simulink model "Communication_rate_control"  (R2025a)
settings: Solver=VariableStepAuto  StartTime=0.0  StopTime=30  RelTol=1e-3
InitFcn:
  | %% Simulation parameters and waypoint trajectory
  | % Initial drone positions.
  | init_0=[0;0;0];
  | d_s=4;
  | init_1=init_0+d_s*[-1;0.1;0];
  | init_2=init_0+d_s*[0.3;-2;0];
  | init_3=init_0+d_s*[0.2;3;0];
  | init_4=init_0+d_s*[4;0.4;0];
  | 
  | Threshold = 1000*ones(45,1);
  | for i=1:9:37
  |     Threshold(i:i+2)=10;
  | end
  | gain_2=1;
  | 
  | % PID controller gains.
  | PID_p=20;
  | PID_i=50;
  | PID_d=0;
  | 
  | % Router queues and background traffic.
  | router_buffer=50;
  | router_bandwith=25;
  | router_init_queue=[2,0,0,0,0];
  | traffic_mean=20;
  | traffic_variance=1;
  | 
  | 
  | % Desired formation offsets.
  | init_f_0=[0;0;0];
  | d_f=1;
  | init_f_1=init_0+d_f*[-1;0;0];
  | init_f_2=init_0+d_f*[0;-1;0];
  | init_f_3=init_0+d_f*[0;1;0];
  | init_f_4=init_0+d_f*[1;0;0];
  | 
  | % Quadrotor mass and inertia.
  | mass = 1.2;
  | Ib   = diag([1.2416 1.2416 2*1.2416]);
  | 
  | % Time grid and waypoint trajectory.
  | Ts        = 0.001;
  | ttot      = 20;
  | tdead     = 10;
  | totalTime = ttot + tdead;
  | Nsamples  = 3000;
  | t_sample  = linspace(0, totalTime, Nsamples);
  | t=t_sample;
  | waypoints = [ ...
  |              0  0 -2 0;
  |              3  4 -5 0;
  |              2  1 -8 0;
  |              0 0 -20 0];
  | 
  | M    = size(waypoints,1);
  | t_wp = linspace(0, ttot, M);
  | 
  | p_d      = zeros(4, Nsamples);
  | dot_p_d  = zeros(4, Nsamples);
  | ddot_p_d = zeros(4, Nsamples);
  | 
  | idx_traj = t_sample <= ttot;
  | t_active = t_sample(idx_traj);
  | 
  | % Build position and yaw splines with zero endpoint velocities.
  | for dim = 1:4
  |     pp  = spline(t_wp, [0, waypoints(:,dim)&apos;, 0]);
  |     pp1 = fnder(pp,1);
  |     pp2 = fnder(pp,2);
  | 
  |     p_d(dim,    idx_traj) = ppval(pp,  t_active);
  |     dot_p_d(dim,idx_traj) = ppval(pp1, t_active);
  |     ddot_p_d(dim,idx_traj)= ppval(pp2, t_active);
  | end
  | 
  | % Hold the final waypoint after the maneuver.
  | last_wp_idx = M;
  | p_d(:, ~idx_traj)      = repmat(waypoints(last_wp_idx,:)&apos;, 1, sum(~idx_traj));
  | dot_p_d(:, ~idx_traj)  = 0;
  | ddot_p_d(:, ~idx_traj) = 0;
  | 
  | % Reference signals used by the Simulink blocks.
  | csi_d      = p_d(1:3,:);
  | psi_d      = p_d(4,:);
  | 
  | dot_csi_d  = dot_p_d(1:3,:);
  | ddot_csi_d = ddot_p_d(1:3,:);
  | dot_psi_d  = dot_p_d(4,:);
  | ddot_psi_d = ddot_p_d(4,:);
  | 
  | pos_0     = waypoints(1,1:3);
  | lin_vel_0 = [0 0 0];
  | w_bb_0    = [0 0 0];
undefined symbols (not defined in the file): A_diacenza, DiscIntNeverNeededParam, K, L
libraries: dspsigops x10, robotcorelib x5, slpidlib x5, dspstat3 x5, uavutilslib x1
(part 1 of 3)
settings Model: Creator=fabioruggiero  LastModifiedBy=Giammo
settings ModelReferenceCC: EnableRefExpFcnMdlSchedulingChecks=on
settings RTWCC: GPUComputeCapability=3.5

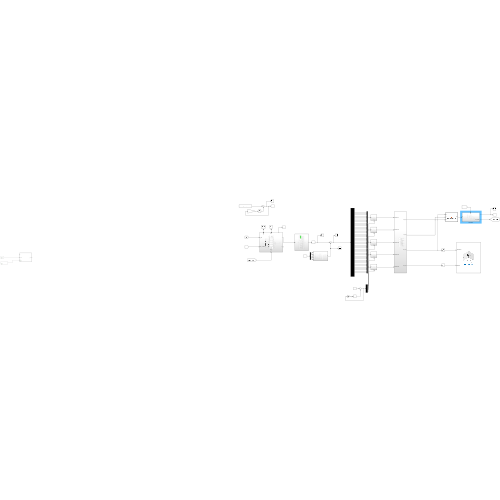
[thumbnail: Simulink's stored preview of the top-level diagram]
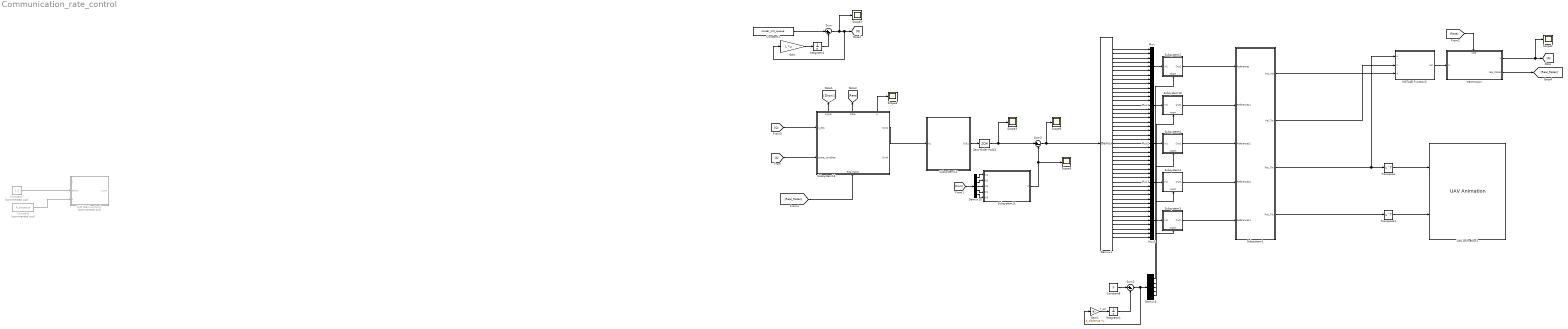
== system Communication_rate_control ==
  Constant : Constant  Commented=on  Value=A_diacenza
  Constant1 : Constant  Value=router_init_queue
  Constant7 : Constant  Commented=on  Value=1.5
  Constant8 : Constant  Value=0
  Demux1 : Demux  Outputs=45
  Demux10 : Demux  Outputs=5
  Demux9 : Demux  Outputs=5
  From : From
  Gain : Gain  Gain=L  Multiplication=Matrix(K*u)
  Gain1 : Gain  Gain=A_diacenza  Multiplication=Matrix(K*u)
  Goto : Goto
  Integrator1 : Integrator
  Integrator2 : Integrator
  MATLAB Function2 : MATLAB Function  TreatAsAtomicUnit=on
  MATLAB Function3 : MATLAB Function  Commented=on  TreatAsAtomicUnit=on
  Mux{,1..3,5} (5 alike) : Mux  Inputs=9
  Scope{1..6} (6 alike) : Scope
      Scope1 settings: ActiveDisplayYMinimum=-19.039927656557538  ActiveDisplayYMaximum=17.096275567841861  DataLoggingVariableName=ScopeData33
      Scope2 settings: ActiveDisplayYMinimum=-0.80480947223759247  ActiveDisplayYMaximum=7.2432852501383342  DataLoggingVariableName=ScopeData34
      Scope3 settings: ActiveDisplayYMinimum=-143.81794768951772  ActiveDisplayYMaximum=72.930943180534939  DataLoggingVariableName=ScopeData22
      Scope4 settings: ActiveDisplayYMinimum=-1  ActiveDisplayYMaximum=1  DataLoggingVariableName=ScopeData10
      Scope5 settings: ActiveDisplayYMinimum=-31.295142586026412  ActiveDisplayYMaximum=31.13864534366818  DataLoggingVariableName=ScopeData26
      Scope6 settings: ActiveDisplayYMinimum=-63.285546446382227  ActiveDisplayYMaximum=68.103390325053155  DataLoggingVariableName=ScopeData30
  Subsystem1 : Subsystem
  Subsystem10 : Subsystem
      settings: PortSchema="{\"entries\":[{\"content\":{\"sides\":[{\"content\":{\"connectorIds\":[\"In1\"]},\"type\":\"ConnectorPlacement.EquallySpacedRectSide\",\"uuid\":\"6e5d8b99-8054-458f-abbe-7e3d6126420c\"},{\"content\":{\"connectorIds\":[\"Out1\"],\"side\":\"RIGHT\"},\"type\":\"ConnectorPlacement.EquallySpacedRectSide\",\"uuid\":\"d8af8c34-1227-4a19-bfdc-b42d943ed13c\"},{\"content\":{\"side\":\"TOP\"},\"type\":\"ConnectorPlacement.EquallySpacedRectSide\",\"uuid\":\"9c10b933-2873-4349-b535-f2af5c16ec70\"},{\"content\":{\"connectorIds\":[\"In2\"],\"side\":\"BOTTOM\"},\"type\":\"ConnectorPlacement.EquallySpacedRectSide\",\"uuid\":\"05be8d01-ed26-4f96-bcb1-0e501cb43bcc\"}]},\"type\":\"ConnectorPlacement.EquallySpacedConnector\",\"uuid\":\"f87e25de-488b-44c6-b2e5-9d22d609821c\"}],\"packageUris\":[\"http://schema.mathworks.com/mf0/Connector/R2020b\"],\"version\":\"1.0\"}"
  Subsystem11 : Subsystem
  Subsystem13 : Subsystem
  Subsystem14 : Subsystem
      settings: PortSchema="{\"entries\":[{\"content\":{\"sides\":[{\"content\":{\"connectorIds\":[\"In1\",\"In2\"]},\"type\":\"ConnectorPlacement.EquallySpacedRectSide\",\"uuid\":\"f1d046dc-675d-4db9-bf29-bca78bce001f\"},{\"content\":{\"connectorIds\":[\"Out1\",\"Out2\"],\"side\":\"RIGHT\"},\"type\":\"ConnectorPlacement.EquallySpacedRectSide\",\"uuid\":\"811f6c37-e862-4f2b-bd7d-8070e0d60dff\"},{\"content\":{\"connectorIds\":[\"Out3\",\"Out4\",\"Out5\"],\"side\":\"TOP\"},\"type\":\"ConnectorPlacement.EquallySpacedRectSide\",\"uuid\":\"cf9e60f1-1ac0-454e-9388-0113fe782dd3\"},{\"content\":{\"connectorIds\":[\"In3\"],\"side\":\"BOTTOM\"},\"type\":\"ConnectorPlacement.EquallySpacedRectSide\",\"uuid\":\"1705a36f-5e80-44a6-ab31-ad29025d66f8\"}]},\"type\":\"ConnectorPlacement.EquallySpacedConnector\",\"uuid\":\"a6589967-962b-441c-ab9d-1a23d8667ece\"}],\"packageUris\":[\"http://schema.mathworks.com/mf0/Connector/R2020b\"],\"version\":\"1.0\"}"
  Subsystem2 : Subsystem
      settings: PortSchema="{\"entries\":[{\"content\":{\"sides\":[{\"content\":{\"connectorIds\":[\"In1\"]},\"type\":\"ConnectorPlacement.EquallySpacedRectSide\",\"uuid\":\"6e5d8b99-8054-458f-abbe-7e3d6126420c\"},{\"content\":{\"connectorIds\":[\"Out1\"],\"side\":\"RIGHT\"},\"type\":\"ConnectorPlacement.EquallySpacedRectSide\",\"uuid\":\"d8af8c34-1227-4a19-bfdc-b42d943ed13c\"},{\"content\":{\"side\":\"TOP\"},\"type\":\"ConnectorPlacement.EquallySpacedRectSide\",\"uuid\":\"9c10b933-2873-4349-b535-f2af5c16ec70\"},{\"content\":{\"connectorIds\":[\"In2\"],\"side\":\"BOTTOM\"},\"type\":\"ConnectorPlacement.EquallySpacedRectSide\",\"uuid\":\"05be8d01-ed26-4f96-bcb1-0e501cb43bcc\"}]},\"type\":\"ConnectorPlacement.EquallySpacedConnector\",\"uuid\":\"f87e25de-488b-44c6-b2e5-9d22d609821c\"}],\"packageUris\":[\"http://schema.mathworks.com/mf0/Connector/R2020b\"],\"version\":\"1.0\"}"
  Subsystem3 : Subsystem
      settings: PortSchema="{\"entries\":[{\"content\":{\"sides\":[{\"content\":{\"connectorIds\":[\"In1\"]},\"type\":\"ConnectorPlacement.EquallySpacedRectSide\",\"uuid\":\"6e5d8b99-8054-458f-abbe-7e3d6126420c\"},{\"content\":{\"connectorIds\":[\"Out1\"],\"side\":\"RIGHT\"},\"type\":\"ConnectorPlacement.EquallySpacedRectSide\",\"uuid\":\"d8af8c34-1227-4a19-bfdc-b42d943ed13c\"},{\"content\":{\"side\":\"TOP\"},\"type\":\"ConnectorPlacement.EquallySpacedRectSide\",\"uuid\":\"9c10b933-2873-4349-b535-f2af5c16ec70\"},{\"content\":{\"connectorIds\":[\"In2\"],\"side\":\"BOTTOM\"},\"type\":\"ConnectorPlacement.EquallySpacedRectSide\",\"uuid\":\"05be8d01-ed26-4f96-bcb1-0e501cb43bcc\"}]},\"type\":\"ConnectorPlacement.EquallySpacedConnector\",\"uuid\":\"f87e25de-488b-44c6-b2e5-9d22d609821c\"}],\"packageUris\":[\"http://schema.mathworks.com/mf0/Connector/R2020b\"],\"version\":\"1.0\"}"
  Subsystem4 : Subsystem
      settings: PortSchema="{\"entries\":[{\"content\":{\"sides\":[{\"content\":{\"connectorIds\":[\"In1\"]},\"type\":\"ConnectorPlacement.EquallySpacedRectSide\",\"uuid\":\"6e5d8b99-8054-458f-abbe-7e3d6126420c\"},{\"content\":{\"connectorIds\":[\"Out1\"],\"side\":\"RIGHT\"},\"type\":\"ConnectorPlacement.EquallySpacedRectSide\",\"uuid\":\"d8af8c34-1227-4a19-bfdc-b42d943ed13c\"},{\"content\":{\"side\":\"TOP\"},\"type\":\"ConnectorPlacement.EquallySpacedRectSide\",\"uuid\":\"9c10b933-2873-4349-b535-f2af5c16ec70\"},{\"content\":{\"connectorIds\":[\"In2\"],\"side\":\"BOTTOM\"},\"type\":\"ConnectorPlacement.EquallySpacedRectSide\",\"uuid\":\"05be8d01-ed26-4f96-bcb1-0e501cb43bcc\"}]},\"type\":\"ConnectorPlacement.EquallySpacedConnector\",\"uuid\":\"f87e25de-488b-44c6-b2e5-9d22d609821c\"}],\"packageUris\":[\"http://schema.mathworks.com/mf0/Connector/R2020b\"],\"version\":\"1.0\"}"
  Subsystem6 : Subsystem
      settings: PortSchema="{\"entries\":[{\"content\":{\"sides\":[{\"content\":{\"connectorIds\":[\"In1\"]},\"type\":\"ConnectorPlacement.EquallySpacedRectSide\",\"uuid\":\"6e5d8b99-8054-458f-abbe-7e3d6126420c\"},{\"content\":{\"connectorIds\":[\"Out1\"],\"side\":\"RIGHT\"},\"type\":\"ConnectorPlacement.EquallySpacedRectSide\",\"uuid\":\"d8af8c34-1227-4a19-bfdc-b42d943ed13c\"},{\"content\":{\"side\":\"TOP\"},\"type\":\"ConnectorPlacement.EquallySpacedRectSide\",\"uuid\":\"9c10b933-2873-4349-b535-f2af5c16ec70\"},{\"content\":{\"connectorIds\":[\"In2\"],\"side\":\"BOTTOM\"},\"type\":\"ConnectorPlacement.EquallySpacedRectSide\",\"uuid\":\"05be8d01-ed26-4f96-bcb1-0e501cb43bcc\"}]},\"type\":\"ConnectorPlacement.EquallySpacedConnector\",\"uuid\":\"f87e25de-488b-44c6-b2e5-9d22d609821c\"}],\"packageUris\":[\"http://schema.mathworks.com/mf0/Connector/R2020b\"],\"version\":\"1.0\"}"
  Sum : Sum  Inputs=|+-
  Sum2 : Sum  Inputs=|+-
  Sum3 : Sum  Inputs=|+-
  Transpose : Math  Operator=transpose
  Transpose1 : Math  Operator=transpose
  UAV Animation1 : uavutilslib/UAV Animation  NumUAV=5  DynamicUAVConfig=off  UAVType=Multirotor  UAVSize=1  UAVColor=[1 0 0]  UAVTrajectoryAlpha=1  InertialZDirection=Down  RotationFormat=Quaternion  DrawMarkers=off  SampleTime=0.01
  Zero-Order Hold1 : ZeroOrderHold  SampleTime=-1
  trasmission : Subsystem
      settings: PortSchema="{\"entries\":[{\"content\":{\"sides\":[{\"content\":{\"connectorIds\":[\"In1\"]},\"type\":\"ConnectorPlacement.EquallySpacedRectSide\",\"uuid\":\"4dfdb4a7-0a88-4bc0-a7e6-6eaded6ab7ea\"},{\"content\":{\"connectorIds\":[\"Out1\",\"Out2\"],\"side\":\"RIGHT\"},\"type\":\"ConnectorPlacement.EquallySpacedRectSide\",\"uuid\":\"9b9e2090-1e21-4d2a-8a8a-73b93d842d99\"},{\"content\":{\"connectorIds\":[\"In2\"],\"side\":\"TOP\"},\"type\":\"ConnectorPlacement.EquallySpacedRectSide\",\"uuid\":\"40eb9426-960b-4b19-8bb6-92ef73d2d0da\"}]},\"type\":\"ConnectorPlacement.EquallySpacedConnector\",\"uuid\":\"8e0959b2-0aca-4b3e-87b3-3e8255b5da73\"}],\"packageUris\":[\"http://schema.mathworks.com/mf0/Connector/R2020b\"],\"version\":\"1.0\"}"
  wires:
  Demux9/5 -> Subsystem3/2(Inport)
  Transpose1/1 -> UAV Animation1/2
  Transpose/1 -> UAV Animation1/1
  Sum2/1 -> Demux9/1, Gain1/1
  Gain1/1 -> Integrator1/1  "P_dot"
  Integrator1/1 -> Sum2/2
  Mux3/1 -> Subsystem4/1(In1)
  Mux/1 -> Subsystem2/1(In1)
  Subsystem2/1(Out1) -> Subsystem1/1(References)
  Demux9/2 -> Subsystem10/2(Inport)
  Subsystem3/1(Out1) -> Subsystem1/5(References4)
  Mux5/1 -> Subsystem3/1(In1)
  Subsystem6/1(Out1) -> Subsystem1/3(References2)
  Mux2/1 -> Subsystem6/1(In1)
  Demux1/1 -> Mux/1
  Demux1/15 -> Mux1/6
  Demux9/1 -> Subsystem2/2(Inport)
  Demux1/23 -> Mux2/5
  Demux1/12 -> Mux1/3
  Demux1/4 -> Mux/4
  Demux1/31 -> Mux3/4
  Demux1/41 -> Mux5/5
  Demux1/19 -> Mux2/1
  Demux1/26 -> Mux2/8
  Demux1/29 -> Mux3/2
  Demux1/34 -> Mux3/7
  Demux1/39 -> Mux5/3
  Demux1/20 -> Mux2/2
  Demux1/38 -> Mux5/2
  Demux1/43 -> Mux5/7
  Demux1/42 -> Mux5/6
  Demux1/30 -> Mux3/3
  Demux1/36 -> Mux3/9
  Demux1/27 -> Mux2/9
  Demux9/4 -> Subsystem4/2(Inport)
  Demux1/22 -> Mux2/4
  Demux1/32 -> Mux3/5
  Demux1/14 -> Mux1/5
  Demux1/13 -> Mux1/4
  Demux1/21 -> Mux2/3
  Demux1/33 -> Mux3/6
  Subsystem1/4(Rot_Tot) -> Transpose1/1
  Demux1/9 -> Mux/9
  Mux1/1 -> Subsystem10/1(In1)
  Demux1/40 -> Mux5/4
  Demux1/3 -> Mux/3
  Demux1/6 -> Mux/6
  Demux1/25 -> Mux2/7
  Demux1/8 -> Mux/8
  Demux1/28 -> Mux3/1
  Demux1/10 -> Mux1/1
  Demux1/7 -> Mux/7
  Demux1/37 -> Mux5/1
  Demux1/11 -> Mux1/2
  Demux1/45 -> Mux5/9
  Demux1/17 -> Mux1/8
  Demux1/35 -> Mux3/8
  Demux1/5 -> Mux/5
  Demux1/44 -> Mux5/8
  Demux1/18 -> Mux1/9
  Demux1/16 -> Mux1/7
  Demux1/2 -> Mux/2
  Constant7/1 -> MATLAB Function3/2(alpha)
  Constant8/1 -> Sum2/1
  Constant/1 -> MATLAB Function3/3(A)
  Subsystem4/1(Out1) -> Subsystem1/4(References3)
  Demux9/3 -> Subsystem6/2(Inport)
  Demux1/24 -> Mux2/6
  Subsystem10/1(Out1) -> Subsystem1/2(References1)
  Subsystem1/3(Pos_Tot) -> MATLAB Function2/1(M), Transpose/1
  Subsystem1/2(Vel_Tot) -> MATLAB Function2/2(V)
  Subsystem1/1(Acc_tot) -> MATLAB Function2/3(A)
  Subsystem11/1(P) -> Scope5/1, Sum3/2
  Demux10/1 -> Subsystem11/1(In1)
  Demux10/2 -> Subsystem11/2(In2)
  Demux10/3 -> Subsystem11/3(In3)
  Demux10/4 -> Subsystem11/4(In4)
  Demux10/5 -> Subsystem11/5(In5)
  [Droni] -> Demux10/1
  Gain/1 -> Integrator2/1
  Constant1/1 -> Sum/1
  trasmission/1(" ") -> Scope1/1, Goto/1
  MATLAB Function2/1(vec) -> trasmission/1(In)
  [Rate] -> trasmission/2(rate)
  [Q] -> Subsystem14/1(q_des)
  From/1 -> Subsystem14/2(state_variables)
  Subsystem14/3(signal) -> [Droni]
  Subsystem14/4(Rate) -> [Rate]
  trasmission/2(real_Rates) -> [Real_Rates]
  [Real_Rates] -> Subsystem14/3(" Real Rates")
  Integrator2/1 -> Sum/2
  Sum/1 -> Scope2/1, Gain/1, [Q]
  Subsystem14/5(q) -> Scope4/1
  Subsystem13/1(Out1) -> Zero-Order Hold1/1
  Zero-Order Hold1/1 -> Scope3/1, Sum3/1
  Sum3/1 -> Demux1/1, Scope6/1
  Subsystem14/1(Out1) -> Subsystem13/1(In1)

== system Communication_rate_control/Subsystem1 ==
  References : Inport
  References1 : Inport  Port=2
  References2 : Inport  Port=3
  References3 : Inport  Port=4
  References4 : Inport  Port=5
  Subsystem : Subsystem
  Subsystem1 : Subsystem
  Subsystem2 : Subsystem
  Subsystem3 : Subsystem
  Subsystem_1 : Subsystem
  Subsystem_2 : Subsystem
  Subsystem_3 : Subsystem
  Subsystem_4 : Subsystem
  Subsystem_5 : Subsystem
  Acc_tot : Outport
  Vel_Tot : Outport  Port=2
  Pos_Tot : Outport  Port=3
  Rot_Tot : Outport  Port=4
  wires:
  References1/1 -> Subsystem_2/1(References)
  References2/1 -> Subsystem_3/1(References)
  References3/1 -> Subsystem_4/1(References)
  References/1 -> Subsystem_1/1(References)
  References4/1 -> Subsystem_5/1(References)
  Subsystem_1/2(Lin Vel) -> Subsystem/1(In1)
  Subsystem_2/2(Lin Vel) -> Subsystem/2(In2)
  Subsystem_3/2(Lin Vel) -> Subsystem/3(In3)
  Subsystem_4/2(Lin Vel) -> Subsystem/4(In4)
  Subsystem_5/2(Lin Vel) -> Subsystem/5(In5)
  Subsystem/1(Out1) -> Vel_Tot/1
  Subsystem_1/3(Lin Pos) -> Subsystem1/1(In1)
  Subsystem_2/3(Lin Pos) -> Subsystem1/2(In2)
  Subsystem_3/3(Lin Pos) -> Subsystem1/3(In3)
  Subsystem_4/3(Lin Pos) -> Subsystem1/4(In4)
  Subsystem_5/3(Lin Pos) -> Subsystem1/5(In5)
  Subsystem1/1(Out1) -> Pos_Tot/1
  Subsystem_1/4(Rotation) -> Subsystem2/1(In1)
  Subsystem_2/4(Rotation) -> Subsystem2/2(In2)
  Subsystem_3/4(Rotation) -> Subsystem2/3(In3)
  Subsystem_4/4(Rotation) -> Subsystem2/4(In4)
  Subsystem_5/4(Rotation) -> Subsystem2/5(In5)
  Subsystem2/1(Out1) -> Rot_Tot/1
  Subsystem_1/1(Lin Acc) -> Subsystem3/1(In1)
  Subsystem_2/1(Lin Acc) -> Subsystem3/2(In2)
  Subsystem_3/1(Lin Acc) -> Subsystem3/3(In3)
  Subsystem_4/1(Lin Acc) -> Subsystem3/4(In4)
  Subsystem_5/1(Lin Acc) -> Subsystem3/5(In5)
  Subsystem3/1(Out1) -> Acc_tot/1

== system Communication_rate_control/Subsystem10 ==
  In1 : Inport
  Inport : Inport  Port=2
  Constant1 : Constant  Value=[0;0;0]
  Demux : Demux  Outputs=9
  Demux1 : Demux  Outputs=3
  Mux : Mux  Inputs=3
  Mux2 : Mux  Inputs=10
  Sum : Sum  Inputs=++|
  Out1 : Outport
  wires:
  Mux2/1 -> Out1/1
  In1/1 -> Demux/1
  Demux/4 -> Mux2/4
  Demux/5 -> Mux2/5
  Demux/6 -> Mux2/6
  Demux/7 -> Mux2/7
  Demux/8 -> Mux2/8
  Demux/9 -> Mux2/9
  Demux/1 -> Mux/1
  Demux/2 -> Mux/2
  Demux/3 -> Mux/3
  Mux/1 -> Sum/2
  Constant1/1 -> Sum/1
  Sum/1 -> Demux1/1
  Demux1/1 -> Mux2/1
  Demux1/2 -> Mux2/2
  Demux1/3 -> Mux2/3
  Inport/1 -> Mux2/10

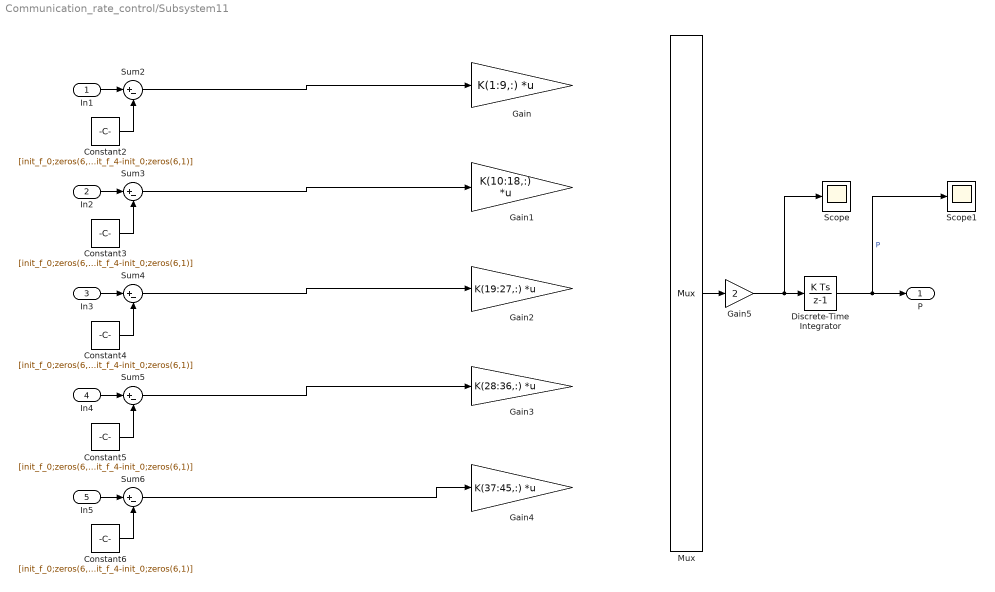
== system Communication_rate_control/Subsystem11 ==
  In1 : Inport
  In2 : Inport  Port=2
  In3 : Inport  Port=3
  In4 : Inport  Port=4
  In5 : Inport  Port=5
  Constant{2..6} (5 alike) : Constant  Value=[init_f_0;zeros(6,1);init_f_1-init_0;zeros(6,1);init_f_2-init_0;zeros(6,1);init_f_3-init_0;zeros(6,1);init_f_4-init_0;zeros(6,1)]
  Discrete-Time Integrator : DiscreteIntegrator  SampleTime=-1  ICPrevOutput=DiscIntNeverNeededParam  ICPrevScaledInput=DiscIntNeverNeededParam
  Gain : Gain  Gain=K(1:9,:)  Multiplication=Matrix(K*u)
  Gain1 : Gain  Gain=K(10:18,:)  Multiplication=Matrix(K*u)
  Gain2 : Gain  Gain=K(19:27,:)  Multiplication=Matrix(K*u)
  Gain3 : Gain  Gain=K(28:36,:)  Multiplication=Matrix(K*u)
  Gain4 : Gain  Gain=K(37:45,:)  Multiplication=Matrix(K*u)
  Gain5 : Gain  Gain=2
  Mux : Mux  Inputs=5
  Scope : Scope
      settings: ActiveDisplayYMinimum=-1  ActiveDisplayYMaximum=1  DataLoggingVariableName=ScopeData27
  Scope1 : Scope
      settings: ActiveDisplayYMinimum=-27.096024824890314  ActiveDisplayYMaximum=25.2419506186057  DataLoggingVariableName=ScopeData28
  Sum{2..6} (5 alike) : Sum  Inputs=|+-
  P : Outport
  wires:
  Discrete-Time Integrator/1 -> Scope1/1, P/1  "P"
  Constant2/1 -> Sum2/2
  Constant3/1 -> Sum3/2
  Constant4/1 -> Sum4/2
  Constant5/1 -> Sum5/2
  Constant6/1 -> Sum6/2
  Mux/1 -> Gain5/1
  In1/1 -> Sum2/1
  In2/1 -> Sum3/1
  In3/1 -> Sum4/1
  In4/1 -> Sum5/1
  In5/1 -> Sum6/1
  Sum6/1 -> Gain4/1
  Sum4/1 -> Gain2/1
  Sum3/1 -> Gain1/1
  Sum2/1 -> Gain/1
  Gain5/1 -> Discrete-Time Integrator/1, Scope/1
  Sum5/1 -> Gain3/1

== system Communication_rate_control/Subsystem13 ==
  In1 : Inport
  Constant{5,10..12} (4 alike) : Constant  Value=0
  Constant3 : Constant  Value=init_1
  Constant4 : Constant  Value=init_3
  Constant6 : Constant  Value=init_4
  Constant9 : Constant  Value=init_2
  Demux : Demux  Outputs=15
  Demux{2..8} (7 alike) : Demux  Outputs=3
  Mux4 : Mux  Inputs=45
  Planner : Subsystem
  Terminator{,1..3} (4 alike) : Terminator
  Out1 : Outport
  wires:
  Demux/10 -> Mux4/34
  Demux6/1 -> Mux4/4
  Mux4/1 -> Out1/1
  Demux6/2 -> Mux4/5
  Demux4/1 -> Mux4/28
  Constant10/1 -> Mux4/13, Mux4/15, Mux4/14
  Demux/15 -> Mux4/45
  Demux3/2 -> Mux4/20
  Demux5/3 -> Mux4/39
  Planner/3(linear_acceleration_des) -> Demux8/1
  Constant9/1 -> Demux3/1
  Demux/3 -> Terminator2/1
  Constant11/1 -> Mux4/31, Mux4/33, Mux4/32
  Demux8/3 -> Mux4/9
  Constant6/1 -> Demux5/1
  Constant12/1 -> Mux4/40, Mux4/41, Mux4/42
  Demux3/1 -> Mux4/19
  Demux6/3 -> Mux4/6
  Demux/6 -> Mux4/18
  Demux8/2 -> Mux4/8
  Demux/1 -> Terminator/1
  Demux5/1 -> Mux4/37
  Demux5/2 -> Mux4/38
  Demux2/3 -> Mux4/3
  In1/1 -> Demux/1
  Demux3/3 -> Mux4/21
  Demux/12 -> Mux4/36
  Demux4/3 -> Mux4/30
  Demux7/2 -> Mux4/11
  Constant5/1 -> Mux4/22, Mux4/24, Mux4/23
  Demux/13 -> Mux4/43
  Constant3/1 -> Demux7/1
  Demux2/2 -> Mux4/2
  Demux/9 -> Mux4/27
  Demux7/3 -> Mux4/12
  Demux/4 -> Mux4/16
  Demux/8 -> Mux4/26
  Planner/4(xb_des) -> Terminator3/1
  Demux/14 -> Mux4/44
  Demux2/1 -> Mux4/1
  Demux/7 -> Mux4/25
  Demux/2 -> Terminator1/1
  Demux/5 -> Mux4/17
  Demux8/1 -> Mux4/7
  Constant4/1 -> Demux4/1
  Demux7/1 -> Mux4/10
  Demux/11 -> Mux4/35
  Planner/2(linear_velocity_des) -> Demux6/1
  Planner/1(position_des) -> Demux2/1
  Demux4/2 -> Mux4/29

== system Communication_rate_control/Subsystem14 ==
  q_des : Inport
  state_variables : Inport  Port=2
  " Real Rates" : Inport  Port=3
  Demux : Demux  Outputs=5
  Mux{6..9} (4 alike) : Mux  Inputs=5
  Subsystem : Subsystem
      settings: PortSchema="{\"entries\":[{\"content\":{\"sides\":[{\"content\":{\"connectorIds\":[\"In1\",\"In2\",\"In3\"]},\"type\":\"ConnectorPlacement.EquallySpacedRectSide\",\"uuid\":\"aabcef1b-4fc2-4bd0-92ff-98af5bae71df\"},{\"content\":{\"connectorIds\":[\"Out1\"],\"side\":\"RIGHT\"},\"type\":\"ConnectorPlacement.EquallySpacedRectSide\",\"uuid\":\"7f481425-bc3c-4684-b5b9-3c38277c27e3\"},{\"content\":{\"connectorIds\":[\"Out2\",\"Out3\",\"Out4\"],\"side\":\"TOP\"},\"type\":\"ConnectorPlacement.EquallySpacedRectSide\",\"uuid\":\"89424cd8-205b-4e4e-84ff-a3a586731ce6\"}]},\"type\":\"ConnectorPlacement.EquallySpacedConnector\",\"uuid\":\"cde5d1e6-587e-462f-b172-cbaeaf24433c\"}],\"packageUris\":[\"http://schema.mathworks.com/mf0/Connector/R2020b\"],\"version\":\"1.0\"}"
  Subsystem5 : Subsystem
      settings: PortSchema="{\"entries\":[{\"content\":{\"sides\":[{\"content\":{\"connectorIds\":[\"In1\",\"In2\",\"In3\"]},\"type\":\"ConnectorPlacement.EquallySpacedRectSide\",\"uuid\":\"aabcef1b-4fc2-4bd0-92ff-98af5bae71df\"},{\"content\":{\"connectorIds\":[\"Out1\"],\"side\":\"RIGHT\"},\"type\":\"ConnectorPlacement.EquallySpacedRectSide\",\"uuid\":\"7f481425-bc3c-4684-b5b9-3c38277c27e3\"},{\"content\":{\"connectorIds\":[\"Out2\",\"Out3\",\"Out4\"],\"side\":\"TOP\"},\"type\":\"ConnectorPlacement.EquallySpacedRectSide\",\"uuid\":\"89424cd8-205b-4e4e-84ff-a3a586731ce6\"}]},\"type\":\"ConnectorPlacement.EquallySpacedConnector\",\"uuid\":\"cde5d1e6-587e-462f-b172-cbaeaf24433c\"}],\"packageUris\":[\"http://schema.mathworks.com/mf0/Connector/R2020b\"],\"version\":\"1.0\"}"
  Subsystem7 : Subsystem
      settings: PortSchema="{\"entries\":[{\"content\":{\"sides\":[{\"content\":{\"connectorIds\":[\"In1\",\"In2\",\"In3\"]},\"type\":\"ConnectorPlacement.EquallySpacedRectSide\",\"uuid\":\"aabcef1b-4fc2-4bd0-92ff-98af5bae71df\"},{\"content\":{\"connectorIds\":[\"Out1\"],\"side\":\"RIGHT\"},\"type\":\"ConnectorPlacement.EquallySpacedRectSide\",\"uuid\":\"7f481425-bc3c-4684-b5b9-3c38277c27e3\"},{\"content\":{\"connectorIds\":[\"Out2\",\"Out3\",\"Out4\"],\"side\":\"TOP\"},\"type\":\"ConnectorPlacement.EquallySpacedRectSide\",\"uuid\":\"89424cd8-205b-4e4e-84ff-a3a586731ce6\"}]},\"type\":\"ConnectorPlacement.EquallySpacedConnector\",\"uuid\":\"cde5d1e6-587e-462f-b172-cbaeaf24433c\"}],\"packageUris\":[\"http://schema.mathworks.com/mf0/Connector/R2020b\"],\"version\":\"1.0\"}"
  Subsystem8 : Subsystem
      settings: PortSchema="{\"entries\":[{\"content\":{\"sides\":[{\"content\":{\"connectorIds\":[\"In1\",\"In2\",\"In3\"]},\"type\":\"ConnectorPlacement.EquallySpacedRectSide\",\"uuid\":\"aabcef1b-4fc2-4bd0-92ff-98af5bae71df\"},{\"content\":{\"connectorIds\":[\"Out1\"],\"side\":\"RIGHT\"},\"type\":\"ConnectorPlacement.EquallySpacedRectSide\",\"uuid\":\"7f481425-bc3c-4684-b5b9-3c38277c27e3\"},{\"content\":{\"connectorIds\":[\"Out2\",\"Out3\",\"Out4\"],\"side\":\"TOP\"},\"type\":\"ConnectorPlacement.EquallySpacedRectSide\",\"uuid\":\"89424cd8-205b-4e4e-84ff-a3a586731ce6\"}]},\"type\":\"ConnectorPlacement.EquallySpacedConnector\",\"uuid\":\"cde5d1e6-587e-462f-b172-cbaeaf24433c\"}],\"packageUris\":[\"http://schema.mathworks.com/mf0/Connector/R2020b\"],\"version\":\"1.0\"}"
  Subsystem9 : Subsystem
      settings: PortSchema="{\"entries\":[{\"content\":{\"sides\":[{\"content\":{\"connectorIds\":[\"In1\",\"In2\",\"In3\"]},\"type\":\"ConnectorPlacement.EquallySpacedRectSide\",\"uuid\":\"aabcef1b-4fc2-4bd0-92ff-98af5bae71df\"},{\"content\":{\"connectorIds\":[\"Out1\"],\"side\":\"RIGHT\"},\"type\":\"ConnectorPlacement.EquallySpacedRectSide\",\"uuid\":\"7f481425-bc3c-4684-b5b9-3c38277c27e3\"},{\"content\":{\"connectorIds\":[\"Out2\",\"Out3\",\"Out4\"],\"side\":\"TOP\"},\"type\":\"ConnectorPlacement.EquallySpacedRectSide\",\"uuid\":\"89424cd8-205b-4e4e-84ff-a3a586731ce6\"}]},\"type\":\"ConnectorPlacement.EquallySpacedConnector\",\"uuid\":\"cde5d1e6-587e-462f-b172-cbaeaf24433c\"}],\"packageUris\":[\"http://schema.mathworks.com/mf0/Connector/R2020b\"],\"version\":\"1.0\"}"
  Out1 : Outport
  Out4 : Outport  Port=2
  signal : Outport  Port=3
  Rate : Outport  Port=4
  q : Outport  Port=5
  wires:
  q_des/1 -> Demux/1
  state_variables/1 -> Subsystem8/3(u), Subsystem9/3(u), Subsystem7/3(u), Subsystem/3(u), Subsystem5/3(u)
  Subsystem/1(ref) -> Mux6/1
  Subsystem7/3(q) -> Mux8/3
  Mux8/1 -> q/1  "q"
  Subsystem5/4(" Rate") -> Mux9/2
  Subsystem/4(" Rate") -> Mux9/1
  Demux/1 -> Subsystem/1(q_des)
  Subsystem7/1(ref) -> Mux6/3
  Subsystem/2("signal ") -> Mux7/1
  Subsystem5/3(q) -> Mux8/2
  Subsystem8/4(" Rate") -> Mux9/4
  Subsystem7/2("signal ") -> Mux7/3
  Mux9/1 -> Rate/1
  Subsystem5/2("signal ") -> Mux7/2
  Subsystem5/1(ref) -> Mux6/2
  Subsystem/3(q) -> Mux8/1
  Subsystem9/3(q) -> Mux8/5
  Subsystem9/2("signal ") -> Mux7/5
  Subsystem8/1(ref) -> Mux6/4
  Subsystem8/3(q) -> Mux8/4
  Subsystem9/1(ref) -> Mux6/5
  Subsystem8/2("signal ") -> Mux7/4
  Subsystem7/4(" Rate") -> Mux9/3
  Subsystem9/4(" Rate") -> Mux9/5
  Mux7/1 -> signal/1
  Mux6/1 -> Out4/1
  Demux/2 -> Subsystem5/1(q_des)
  Demux/3 -> Subsystem7/1(q_des)
  Demux/4 -> Subsystem8/1(q_des)
  Demux/5 -> Subsystem9/1(q_des)
  " Real Rates"/1 -> Subsystem8/2(" Real Rates"), Subsystem9/2(" Real Rates"), Subsystem7/2(" Real Rates"), Subsystem/2(" Real Rates"), Subsystem5/2(" Real Rates")

== system Communication_rate_control/Subsystem2 ==
  In1 : Inport
  Inport : Inport  Port=2
  Constant1 : Constant  Value=[0;0;0]
  Demux : Demux  Outputs=9
  Demux1 : Demux  Outputs=3
  Mux : Mux  Inputs=3
  Mux2 : Mux  Inputs=10
  Sum : Sum  Inputs=++|
  Out1 : Outport
  wires:
  Mux2/1 -> Out1/1
  In1/1 -> Demux/1
  Demux/4 -> Mux2/4
  Demux/5 -> Mux2/5
  Demux/6 -> Mux2/6
  Demux/7 -> Mux2/7
  Demux/8 -> Mux2/8
  Demux/9 -> Mux2/9
  Demux/1 -> Mux/1
  Demux/2 -> Mux/2
  Demux/3 -> Mux/3
  Mux/1 -> Sum/2
  Constant1/1 -> Sum/1
  Sum/1 -> Demux1/1
  Demux1/1 -> Mux2/1
  Demux1/2 -> Mux2/2
  Demux1/3 -> Mux2/3
  Inport/1 -> Mux2/10

== system Communication_rate_control/Subsystem3 ==
  In1 : Inport
  Inport : Inport  Port=2
  Constant1 : Constant  Value=[0;0;0]
  Demux : Demux  Outputs=9
  Demux1 : Demux  Outputs=3
  Mux : Mux  Inputs=3
  Mux2 : Mux  Inputs=10
  Sum : Sum  Inputs=++|
  Out1 : Outport
  wires:
  Mux2/1 -> Out1/1
  In1/1 -> Demux/1
  Demux/4 -> Mux2/4
  Demux/5 -> Mux2/5
  Demux/6 -> Mux2/6
  Demux/7 -> Mux2/7
  Demux/8 -> Mux2/8
  Demux/9 -> Mux2/9
  Demux/1 -> Mux/1
  Demux/2 -> Mux/2
  Demux/3 -> Mux/3
  Mux/1 -> Sum/2
  Constant1/1 -> Sum/1
  Sum/1 -> Demux1/1
  Demux1/1 -> Mux2/1
  Demux1/2 -> Mux2/2
  Demux1/3 -> Mux2/3
  Inport/1 -> Mux2/10

== system Communication_rate_control/Subsystem4 ==
  In1 : Inport
  Inport : Inport  Port=2
  Constant1 : Constant  Value=[0;0;0]
  Demux : Demux  Outputs=9
  Demux1 : Demux  Outputs=3
  Mux : Mux  Inputs=3
  Mux2 : Mux  Inputs=10
  Sum : Sum  Inputs=++|
  Out1 : Outport
  wires:
  Mux2/1 -> Out1/1
  In1/1 -> Demux/1
  Demux/4 -> Mux2/4
  Demux/5 -> Mux2/5
  Demux/6 -> Mux2/6
  Demux/7 -> Mux2/7
  Demux/8 -> Mux2/8
  Demux/9 -> Mux2/9
  Demux/1 -> Mux/1
  Demux/2 -> Mux/2
  Demux/3 -> Mux/3
  Mux/1 -> Sum/2
  Constant1/1 -> Sum/1
  Sum/1 -> Demux1/1
  Demux1/1 -> Mux2/1
  Demux1/2 -> Mux2/2
  Demux1/3 -> Mux2/3
  Inport/1 -> Mux2/10

== system Communication_rate_control/Subsystem6 ==
  In1 : Inport
  Inport : Inport  Port=2
  Constant1 : Constant  Value=[0;0;0]
  Demux : Demux  Outputs=9
  Demux1 : Demux  Outputs=3
  Mux : Mux  Inputs=3
  Mux2 : Mux  Inputs=10
  Sum : Sum  Inputs=++|
  Out1 : Outport
  wires:
  Mux2/1 -> Out1/1
  In1/1 -> Demux/1
  Demux/4 -> Mux2/4
  Demux/5 -> Mux2/5
  Demux/6 -> Mux2/6
  Demux/7 -> Mux2/7
  Demux/8 -> Mux2/8
  Demux/9 -> Mux2/9
  Demux/1 -> Mux/1
  Demux/2 -> Mux/2
  Demux/3 -> Mux/3
  Mux/1 -> Sum/2
  Constant1/1 -> Sum/1
  Sum/1 -> Demux1/1
  Demux1/1 -> Mux2/1
  Demux1/2 -> Mux2/2
  Demux1/3 -> Mux2/3
  Inport/1 -> Mux2/10

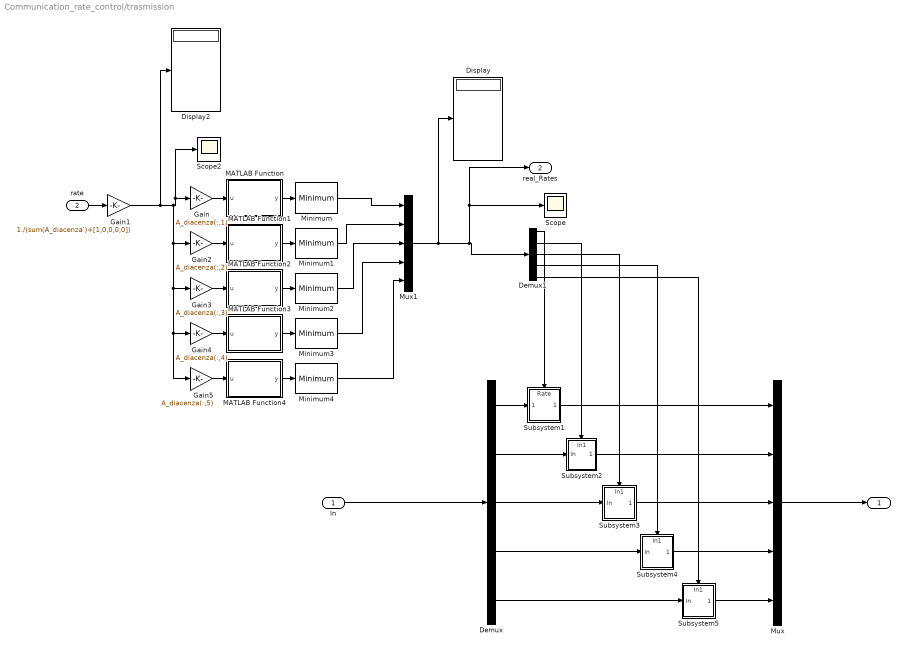
== system Communication_rate_control/trasmission ==
  In : Inport
  rate : Inport  Port=2
  Demux : Demux  Outputs=5
  Demux1 : Demux  Outputs=5
  Display : Display
  Display2 : Display
  Gain : Gain  Gain=A_diacenza(:,1)
  Gain1 : Gain  Gain=1./(sum(A_diacenza')+[1,0,0,0,0])
  Gain2 : Gain  Gain=A_diacenza(:,2)
  Gain3 : Gain  Gain=A_diacenza(:,3)
  Gain4 : Gain  Gain=A_diacenza(:,4)
  Gain5 : Gain  Gain=A_diacenza(:,5)
  MATLAB Function : MATLAB Function  TreatAsAtomicUnit=on
  MATLAB Function1 : MATLAB Function  TreatAsAtomicUnit=on
  MATLAB Function2 : MATLAB Function  TreatAsAtomicUnit=on
  MATLAB Function3 : MATLAB Function  TreatAsAtomicUnit=on
  MATLAB Function4 : MATLAB Function  TreatAsAtomicUnit=on
  Minimum{,1..4} (5 alike) : dspstat3/Minimum  operation=minimum  fcn=Value  indexBase=One  operateOver=Each column  Dimension=1  InputProcessing=Columns as channels (frame based)  reset=None  roiEnable=off  roiType=Rectangles  roiPortion=Entire ROI  roiOutput=Individual statistics for each ROI  roiFlag=off  roundingMode=Floor  overflowMode=off
      settings: LibrarySourceBlock=dsphdlsupportstat/Minimum
  Mux : Mux  Inputs=5
  Mux1 : Mux  Inputs=5
  Scope : Scope
      settings: ActiveDisplayYMinimum=-12.498378799500772  ActiveDisplayYMaximum=112.48540919550697  DataLoggingVariableName=ScopeData11
  Scope2 : Scope
      settings: ActiveDisplayYMinimum=-54.064201882682504  ActiveDisplayYMaximum=119.71379613633677  DataLoggingVariableName=ScopeData24
  Subsystem1 : Subsystem
      settings: PortSchema="{\"entries\":[{\"content\":{\"sides\":[{\"content\":{\"connectorIds\":[\"In1\"]},\"type\":\"ConnectorPlacement.EquallySpacedRectSide\",\"uuid\":\"f5d1fedb-69fc-4b21-9d1f-1508050d7e45\"},{\"content\":{\"connectorIds\":[\"Out1\"],\"side\":\"RIGHT\"},\"type\":\"ConnectorPlacement.EquallySpacedRectSide\",\"uuid\":\"ccd2a0b1-945e-4f3a-9247-4e948aabf2d0\"},{\"content\":{\"connectorIds\":[\"In2\"],\"side\":\"TOP\"},\"type\":\"ConnectorPlacement.EquallySpacedRectSide\",\"uuid\":\"67187460-0f76-4d6b-9cd2-8d40c3ab2945\"}]},\"type\":\"ConnectorPlacement.EquallySpacedConnector\",\"uuid\":\"895ba139-3164-4608-95d1-7f809c1b8c13\"}],\"packageUris\":[\"http://schema.mathworks.com/mf0/Connector/R2020b\"],\"version\":\"1.0\"}"
  Subsystem2 : Subsystem
      settings: PortSchema="{\"entries\":[{\"content\":{\"sides\":[{\"content\":{\"connectorIds\":[\"In1\"]},\"type\":\"ConnectorPlacement.EquallySpacedRectSide\",\"uuid\":\"f5d1fedb-69fc-4b21-9d1f-1508050d7e45\"},{\"content\":{\"connectorIds\":[\"Out1\"],\"side\":\"RIGHT\"},\"type\":\"ConnectorPlacement.EquallySpacedRectSide\",\"uuid\":\"ccd2a0b1-945e-4f3a-9247-4e948aabf2d0\"},{\"content\":{\"connectorIds\":[\"In2\"],\"side\":\"TOP\"},\"type\":\"ConnectorPlacement.EquallySpacedRectSide\",\"uuid\":\"67187460-0f76-4d6b-9cd2-8d40c3ab2945\"}]},\"type\":\"ConnectorPlacement.EquallySpacedConnector\",\"uuid\":\"895ba139-3164-4608-95d1-7f809c1b8c13\"}],\"packageUris\":[\"http://schema.mathworks.com/mf0/Connector/R2020b\"],\"version\":\"1.0\"}"
  Subsystem3 : Subsystem
      settings: PortSchema="{\"entries\":[{\"content\":{\"sides\":[{\"content\":{\"connectorIds\":[\"In1\"]},\"type\":\"ConnectorPlacement.EquallySpacedRectSide\",\"uuid\":\"f5d1fedb-69fc-4b21-9d1f-1508050d7e45\"},{\"content\":{\"connectorIds\":[\"Out1\"],\"side\":\"RIGHT\"},\"type\":\"ConnectorPlacement.EquallySpacedRectSide\",\"uuid\":\"ccd2a0b1-945e-4f3a-9247-4e948aabf2d0\"},{\"content\":{\"connectorIds\":[\"In2\"],\"side\":\"TOP\"},\"type\":\"ConnectorPlacement.EquallySpacedRectSide\",\"uuid\":\"67187460-0f76-4d6b-9cd2-8d40c3ab2945\"}]},\"type\":\"ConnectorPlacement.EquallySpacedConnector\",\"uuid\":\"895ba139-3164-4608-95d1-7f809c1b8c13\"}],\"packageUris\":[\"http://schema.mathworks.com/mf0/Connector/R2020b\"],\"version\":\"1.0\"}"
  Subsystem4 : Subsystem
      settings: PortSchema="{\"entries\":[{\"content\":{\"sides\":[{\"content\":{\"connectorIds\":[\"In1\"]},\"type\":\"ConnectorPlacement.EquallySpacedRectSide\",\"uuid\":\"f5d1fedb-69fc-4b21-9d1f-1508050d7e45\"},{\"content\":{\"connectorIds\":[\"Out1\"],\"side\":\"RIGHT\"},\"type\":\"ConnectorPlacement.EquallySpacedRectSide\",\"uuid\":\"ccd2a0b1-945e-4f3a-9247-4e948aabf2d0\"},{\"content\":{\"connectorIds\":[\"In2\"],\"side\":\"TOP\"},\"type\":\"ConnectorPlacement.EquallySpacedRectSide\",\"uuid\":\"67187460-0f76-4d6b-9cd2-8d40c3ab2945\"}]},\"type\":\"ConnectorPlacement.EquallySpacedConnector\",\"uuid\":\"895ba139-3164-4608-95d1-7f809c1b8c13\"}],\"packageUris\":[\"http://schema.mathworks.com/mf0/Connector/R2020b\"],\"version\":\"1.0\"}"
  Subsystem5 : Subsystem
      settings: PortSchema="{\"entries\":[{\"content\":{\"sides\":[{\"content\":{\"connectorIds\":[\"In1\"]},\"type\":\"ConnectorPlacement.EquallySpacedRectSide\",\"uuid\":\"f5d1fedb-69fc-4b21-9d1f-1508050d7e45\"},{\"content\":{\"connectorIds\":[\"Out1\"],\"side\":\"RIGHT\"},\"type\":\"ConnectorPlacement.EquallySpacedRectSide\",\"uuid\":\"ccd2a0b1-945e-4f3a-9247-4e948aabf2d0\"},{\"content\":{\"connectorIds\":[\"In2\"],\"side\":\"TOP\"},\"type\":\"ConnectorPlacement.EquallySpacedRectSide\",\"uuid\":\"67187460-0f76-4d6b-9cd2-8d40c3ab2945\"}]},\"type\":\"ConnectorPlacement.EquallySpacedConnector\",\"uuid\":\"895ba139-3164-4608-95d1-7f809c1b8c13\"}],\"packageUris\":[\"http://schema.mathworks.com/mf0/Connector/R2020b\"],\"version\":\"1.0\"}"
  " " : Outport
  real_Rates : Outport  Port=2
  wires:
  In/1 -> Demux/1
  Mux/1 -> " "/1
  Demux1/1 -> Subsystem1/2(Rate)
  Demux1/2 -> Subsystem2/2(In1)
  Demux1/3 -> Subsystem3/2(In1)
  Demux1/4 -> Subsystem4/2(In1)
  Demux1/5 -> Subsystem5/2(In1)
  Demux/1 -> Subsystem1/1(Data)
  Demux/2 -> Subsystem2/1(In)
  Subsystem1/1("Samples ") -> Mux/1
  Subsystem2/1(" ") -> Mux/2
  Demux/3 -> Subsystem3/1(In)
  Demux/4 -> Subsystem4/1(In)
  Subsystem3/1(" ") -> Mux/3
  Subsystem4/1(" ") -> Mux/4
  Subsystem5/1(" ") -> Mux/5
  Demux/5 -> Subsystem5/1(In)
  rate/1 -> Gain1/1
  Gain1/1 -> Display2/1, Gain2/1, Gain3/1, Gain5/1, Gain4/1, Gain/1, Scope2/1
  Minimum/1 -> Mux1/1
  Minimum1/1 -> Mux1/2
  Minimum2/1 -> Mux1/3
  Minimum3/1 -> Mux1/4
  Minimum4/1 -> Mux1/5
  Mux1/1 -> Display/1, Scope/1, real_Rates/1, Demux1/1
  Gain/1 -> MATLAB Function/1(u)
  MATLAB Function/1(y) -> Minimum/1
  Gain2/1 -> MATLAB Function1/1(u)
  Gain3/1 -> MATLAB Function2/1(u)
  Gain4/1 -> MATLAB Function3/1(u)
  Gain5/1 -> MATLAB Function4/1(u)
  MATLAB Function4/1(y) -> Minimum4/1
  MATLAB Function3/1(y) -> Minimum3/1
  MATLAB Function2/1(y) -> Minimum2/1
  MATLAB Function1/1(y) -> Minimum1/1

== system Communication_rate_control/Subsystem1/Subsystem ==
  In1 : Inport
  In2 : Inport  Port=2
  In3 : Inport  Port=3
  In4 : Inport  Port=4
  In5 : Inport  Port=5
  Matrix Concatenate2 : Concatenate  NumInputs=5  Mode=Multidimensional array  ConcatenateDimension=2
  Out1 : Outport
  wires:
  In3/1 -> Matrix Concatenate2/3
  In5/1 -> Matrix Concatenate2/5
  In4/1 -> Matrix Concatenate2/4
  In2/1 -> Matrix Concatenate2/2
  In1/1 -> Matrix Concatenate2/1
  Matrix Concatenate2/1 -> Out1/1

== system Communication_rate_control/Subsystem1/Subsystem1 ==
  In1 : Inport
  In2 : Inport  Port=2
  In3 : Inport  Port=3
  In4 : Inport  Port=4
  In5 : Inport  Port=5
  Matrix Concatenate : Concatenate  NumInputs=5  Mode=Multidimensional array  ConcatenateDimension=2
  Out1 : Outport
  wires:
  In5/1 -> Matrix Concatenate/5
  Matrix Concatenate/1 -> Out1/1
  In2/1 -> Matrix Concatenate/2
  In3/1 -> Matrix Concatenate/3
  In1/1 -> Matrix Concatenate/1
  In4/1 -> Matrix Concatenate/4

== system Communication_rate_control/Subsystem1/Subsystem2 ==
  In1 : Inport
  In2 : Inport  Port=2
  In3 : Inport  Port=3
  In4 : Inport  Port=4
  In5 : Inport  Port=5
  Matrix Concatenate1 : Concatenate  NumInputs=5  Mode=Multidimensional array  ConcatenateDimension=2
  Out1 : Outport
  wires:
  In4/1 -> Matrix Concatenate1/4
  In2/1 -> Matrix Concatenate1/2
  In5/1 -> Matrix Concatenate1/5
  Matrix Concatenate1/1 -> Out1/1
  In1/1 -> Matrix Concatenate1/1
  In3/1 -> Matrix Concatenate1/3

== system Communication_rate_control/Subsystem1/Subsystem3 ==
  In1 : Inport
  In2 : Inport  Port=2
  In3 : Inport  Port=3
  In4 : Inport  Port=4
  In5 : Inport  Port=5
  Matrix Concatenate3 : Concatenate  NumInputs=5  Mode=Multidimensional array  ConcatenateDimension=2
  Out1 : Outport
  wires:
  In5/1 -> Matrix Concatenate3/5
  Matrix Concatenate3/1 -> Out1/1
  In3/1 -> Matrix Concatenate3/3
  In4/1 -> Matrix Concatenate3/4
  In2/1 -> Matrix Concatenate3/2
  In1/1 -> Matrix Concatenate3/1

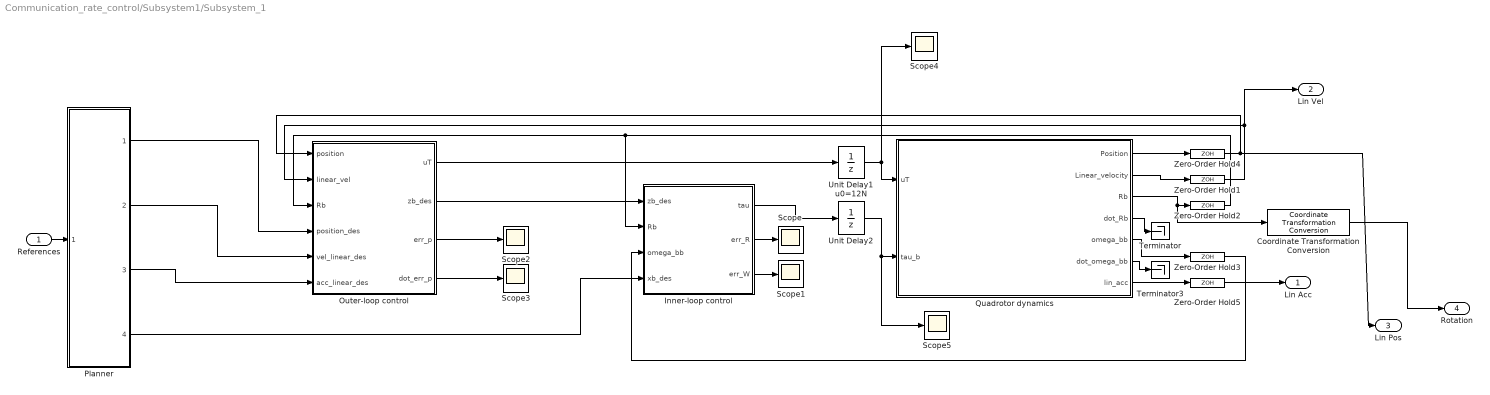
== system Communication_rate_control/Subsystem1/Subsystem_1 ==
  References : Inport
  Coordinate Transformation Conversion : robotcorelib/Coordinate Transformation Conversion  InputRepresentation=Rotation Matrix  InputEulerSequence=ZYX  ShowTrVecInputPort=on  OutputRepresentation=Quaternion  OutputEulerSequence=ZYX  ShowTrVecOutputPort=on  SimulateUsing=Interpreted execution
  Inner-loop control : Subsystem
  Outer-loop control : MATLAB Function  TreatAsAtomicUnit=on
  Planner : Subsystem
  Quadrotor dynamics : Subsystem
  Scope{,1..5} (6 alike) : Scope
      Scope settings: ActiveDisplayYMinimum=-1.2E-5  ActiveDisplayYMaximum=1.2E-5
      Scope1 settings: ActiveDisplayYMinimum=-1.2E-5  ActiveDisplayYMaximum=1.2E-5
      Scope2 settings: ActiveDisplayYMinimum=-3.9E-5  ActiveDisplayYMaximum=1.1E-5  DataLoggingVariableName=ScopeData2
      Scope3 settings: ActiveDisplayYMinimum=-0.00022  ActiveDisplayYMaximum=0.00011  DataLoggingVariableName=ScopeData3
      Scope4 settings: ActiveDisplayYMinimum=11.66748  ActiveDisplayYMaximum=12.03695  DataLoggingVariableName=ScopeData4
      Scope5 settings: ActiveDisplayYMinimum=-0.02035  ActiveDisplayYMaximum=0.02036  DataLoggingVariableName=ScopeData5
  Terminator : Terminator
  Terminator3 : Terminator
  Unit Delay1 u0=12N : UnitDelay  InitialCondition=12  SampleTime=Ts
  Unit Delay2 : UnitDelay  InitialCondition=[0 0 0]  SampleTime=Ts
  Zero-Order Hold{1..5} (5 alike) : ZeroOrderHold  SampleTime=Ts
  Lin Acc : Outport
  Lin Vel : Outport  Port=2
  Lin Pos : Outport  Port=3
  Rotation : Outport  Port=4
  wires:
  Zero-Order Hold5/1 -> Lin Acc/1
  Quadrotor dynamics/7(lin_acc) -> Zero-Order Hold5/1
  Planner/1(position_des) -> Outer-loop control/4(position_des)
  Quadrotor dynamics/1(Position) -> Zero-Order Hold4/1
  Quadrotor dynamics/3(Rb) -> Zero-Order Hold2/1, Coordinate Transformation Conversion/1
  Quadrotor dynamics/4(dot_Rb) -> Terminator/1
  Planner/4(xb_des) -> Inner-loop control/4(xb_des)
  Inner-loop control/1(tau) -> Unit Delay2/1
  Planner/2(linear_velocity_des) -> Outer-loop control/5(vel_linear_des)
  Quadrotor dynamics/2(Linear_velocity) -> Zero-Order Hold1/1
  Quadrotor dynamics/6(dot_omega_bb) -> Terminator3/1
  Outer-loop control/3(err_p) -> Scope2/1
  Coordinate Transformation Conversion/1 -> Rotation/1
  Quadrotor dynamics/5(omega_bb) -> Zero-Order Hold3/1
  Zero-Order Hold2/1 -> Inner-loop control/2(Rb), Outer-loop control/3(Rb)
  References/1 -> Planner/1(References)
  Planner/3(linear_acceleration_des) -> Outer-loop control/6(acc_linear_des)
  Inner-loop control/3(err_W) -> Scope1/1
  Outer-loop control/2(zb_des) -> Inner-loop control/1(zb_des)
  Inner-loop control/2(err_R) -> Scope/1
  Outer-loop control/1(uT) -> Unit Delay1 u0=12N/1
  Unit Delay2/1 -> Quadrotor dynamics/2(tau_b), Scope5/1
  Zero-Order Hold3/1 -> Inner-loop control/3(omega_bb)
  Unit Delay1 u0=12N/1 -> Scope4/1, Quadrotor dynamics/1(uT)
  Outer-loop control/4(dot_err_p) -> Scope3/1
  Zero-Order Hold1/1 -> Outer-loop control/2(linear_vel), Lin Vel/1
  Zero-Order Hold4/1 -> Outer-loop control/1(position), Lin Pos/1

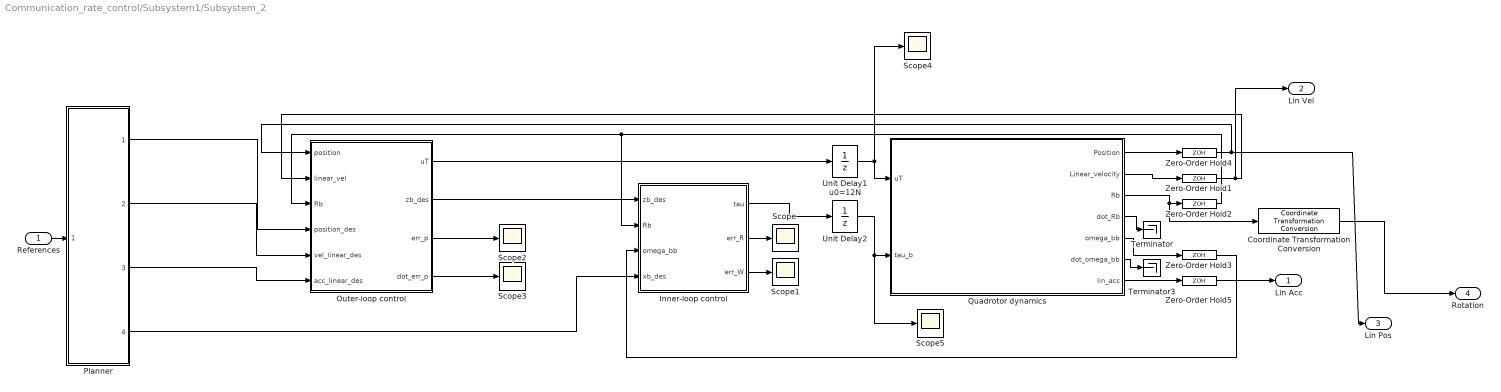
== system Communication_rate_control/Subsystem1/Subsystem_2 ==
  References : Inport
  Coordinate Transformation Conversion : robotcorelib/Coordinate Transformation Conversion  InputRepresentation=Rotation Matrix  InputEulerSequence=ZYX  ShowTrVecInputPort=on  OutputRepresentation=Quaternion  OutputEulerSequence=ZYX  ShowTrVecOutputPort=on  SimulateUsing=Interpreted execution
  Inner-loop control : Subsystem
  Outer-loop control : MATLAB Function  TreatAsAtomicUnit=on
  Planner : Subsystem
  Quadrotor dynamics : Subsystem
  Scope{,1..5} (6 alike) : Scope
      Scope settings: ActiveDisplayYMinimum=-1.2E-5  ActiveDisplayYMaximum=1.2E-5
      Scope1 settings: ActiveDisplayYMinimum=-1.2E-5  ActiveDisplayYMaximum=1.2E-5
      Scope2 settings: ActiveDisplayYMinimum=-3.9E-5  ActiveDisplayYMaximum=1.1E-5  DataLoggingVariableName=ScopeData2
      Scope3 settings: ActiveDisplayYMinimum=-0.00022  ActiveDisplayYMaximum=0.00011  DataLoggingVariableName=ScopeData3
      Scope4 settings: ActiveDisplayYMinimum=11.66748  ActiveDisplayYMaximum=12.03695  DataLoggingVariableName=ScopeData4
      Scope5 settings: ActiveDisplayYMinimum=-0.02035  ActiveDisplayYMaximum=0.02036  DataLoggingVariableName=ScopeData5
  Terminator : Terminator
  Terminator3 : Terminator
  Unit Delay1 u0=12N : UnitDelay  InitialCondition=12  SampleTime=Ts
  Unit Delay2 : UnitDelay  InitialCondition=[0 0 0]  SampleTime=Ts
  Zero-Order Hold{1..5} (5 alike) : ZeroOrderHold  SampleTime=Ts
  Lin Acc : Outport
  Lin Vel : Outport  Port=2
  Lin Pos : Outport  Port=3
  Rotation : Outport  Port=4
  wires:
  Zero-Order Hold5/1 -> Lin Acc/1
  Quadrotor dynamics/7(lin_acc) -> Zero-Order Hold5/1
  Planner/1(position_des) -> Outer-loop control/4(position_des)
  Quadrotor dynamics/1(Position) -> Zero-Order Hold4/1
  Quadrotor dynamics/3(Rb) -> Zero-Order Hold2/1, Coordinate Transformation Conversion/1
  Quadrotor dynamics/4(dot_Rb) -> Terminator/1
  Planner/4(xb_des) -> Inner-loop control/4(xb_des)
  Inner-loop control/1(tau) -> Unit Delay2/1
  Planner/2(linear_velocity_des) -> Outer-loop control/5(vel_linear_des)
  Quadrotor dynamics/2(Linear_velocity) -> Zero-Order Hold1/1
  Quadrotor dynamics/6(dot_omega_bb) -> Terminator3/1
  Outer-loop control/3(err_p) -> Scope2/1
  Coordinate Transformation Conversion/1 -> Rotation/1
  Quadrotor dynamics/5(omega_bb) -> Zero-Order Hold3/1
  Zero-Order Hold2/1 -> Inner-loop control/2(Rb), Outer-loop control/3(Rb)
  References/1 -> Planner/1(References)
  Planner/3(linear_acceleration_des) -> Outer-loop control/6(acc_linear_des)
  Inner-loop control/3(err_W) -> Scope1/1
  Outer-loop control/2(zb_des) -> Inner-loop control/1(zb_des)
  Inner-loop control/2(err_R) -> Scope/1
  Outer-loop control/1(uT) -> Unit Delay1 u0=12N/1
  Unit Delay2/1 -> Quadrotor dynamics/2(tau_b), Scope5/1
  Zero-Order Hold3/1 -> Inner-loop control/3(omega_bb)
  Unit Delay1 u0=12N/1 -> Scope4/1, Quadrotor dynamics/1(uT)
  Outer-loop control/4(dot_err_p) -> Scope3/1
  Zero-Order Hold1/1 -> Outer-loop control/2(linear_vel), Lin Vel/1
  Zero-Order Hold4/1 -> Outer-loop control/1(position), Lin Pos/1

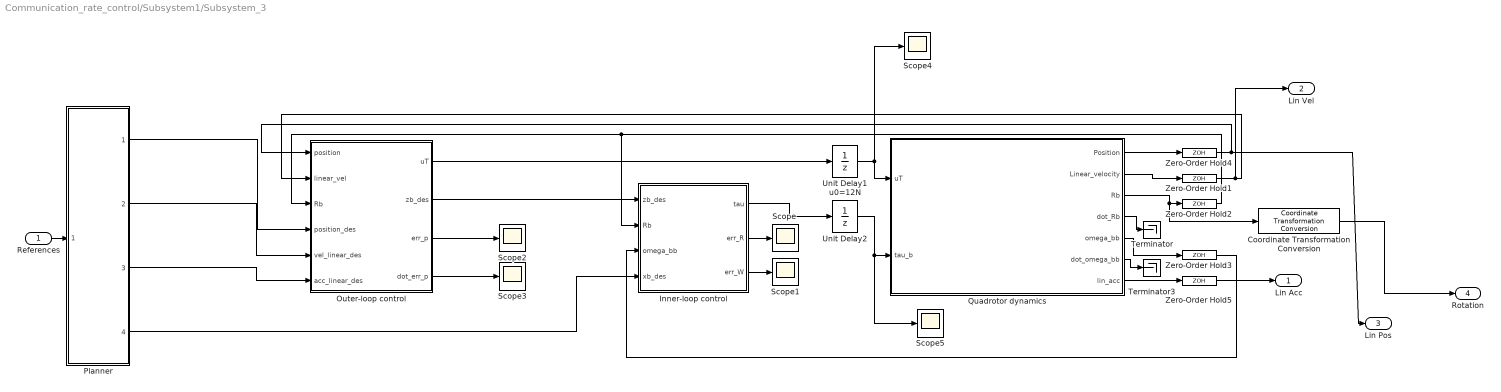
== system Communication_rate_control/Subsystem1/Subsystem_3 ==
  References : Inport
  Coordinate Transformation Conversion : robotcorelib/Coordinate Transformation Conversion  InputRepresentation=Rotation Matrix  InputEulerSequence=ZYX  ShowTrVecInputPort=on  OutputRepresentation=Quaternion  OutputEulerSequence=ZYX  ShowTrVecOutputPort=on  SimulateUsing=Interpreted execution
  Inner-loop control : Subsystem
  Outer-loop control : MATLAB Function  TreatAsAtomicUnit=on
  Planner : Subsystem
  Quadrotor dynamics : Subsystem
  Scope{,1..5} (6 alike) : Scope
      Scope settings: ActiveDisplayYMinimum=-1.2E-5  ActiveDisplayYMaximum=1.2E-5
      Scope1 settings: ActiveDisplayYMinimum=-1.2E-5  ActiveDisplayYMaximum=1.2E-5
      Scope2 settings: ActiveDisplayYMinimum=-3.9E-5  ActiveDisplayYMaximum=1.1E-5  DataLoggingVariableName=ScopeData2
      Scope3 settings: ActiveDisplayYMinimum=-0.00022  ActiveDisplayYMaximum=0.00011  DataLoggingVariableName=ScopeData3
      Scope4 settings: ActiveDisplayYMinimum=11.66748  ActiveDisplayYMaximum=12.03695  DataLoggingVariableName=ScopeData4
      Scope5 settings: ActiveDisplayYMinimum=-0.02035  ActiveDisplayYMaximum=0.02036  DataLoggingVariableName=ScopeData5
  Terminator : Terminator
  Terminator3 : Terminator
  Unit Delay1 u0=12N : UnitDelay  InitialCondition=12  SampleTime=Ts
  Unit Delay2 : UnitDelay  InitialCondition=[0 0 0]  SampleTime=Ts
  Zero-Order Hold{1..5} (5 alike) : ZeroOrderHold  SampleTime=Ts
  Lin Acc : Outport
  Lin Vel : Outport  Port=2
  Lin Pos : Outport  Port=3
  Rotation : Outport  Port=4
  wires:
  Zero-Order Hold5/1 -> Lin Acc/1
  Quadrotor dynamics/7(lin_acc) -> Zero-Order Hold5/1
  Planner/1(position_des) -> Outer-loop control/4(position_des)
  Quadrotor dynamics/1(Position) -> Zero-Order Hold4/1
  Quadrotor dynamics/3(Rb) -> Zero-Order Hold2/1, Coordinate Transformation Conversion/1
  Quadrotor dynamics/4(dot_Rb) -> Terminator/1
  Planner/4(xb_des) -> Inner-loop control/4(xb_des)
  Inner-loop control/1(tau) -> Unit Delay2/1
  Planner/2(linear_velocity_des) -> Outer-loop control/5(vel_linear_des)
  Quadrotor dynamics/2(Linear_velocity) -> Zero-Order Hold1/1
  Quadrotor dynamics/6(dot_omega_bb) -> Terminator3/1
  Outer-loop control/3(err_p) -> Scope2/1
  Coordinate Transformation Conversion/1 -> Rotation/1
  Quadrotor dynamics/5(omega_bb) -> Zero-Order Hold3/1
  Zero-Order Hold2/1 -> Inner-loop control/2(Rb), Outer-loop control/3(Rb)
  References/1 -> Planner/1(References)
  Planner/3(linear_acceleration_des) -> Outer-loop control/6(acc_linear_des)
  Inner-loop control/3(err_W) -> Scope1/1
  Outer-loop control/2(zb_des) -> Inner-loop control/1(zb_des)
  Inner-loop control/2(err_R) -> Scope/1
  Outer-loop control/1(uT) -> Unit Delay1 u0=12N/1
  Unit Delay2/1 -> Quadrotor dynamics/2(tau_b), Scope5/1
  Zero-Order Hold3/1 -> Inner-loop control/3(omega_bb)
  Unit Delay1 u0=12N/1 -> Scope4/1, Quadrotor dynamics/1(uT)
  Outer-loop control/4(dot_err_p) -> Scope3/1
  Zero-Order Hold1/1 -> Outer-loop control/2(linear_vel), Lin Vel/1
  Zero-Order Hold4/1 -> Outer-loop control/1(position), Lin Pos/1

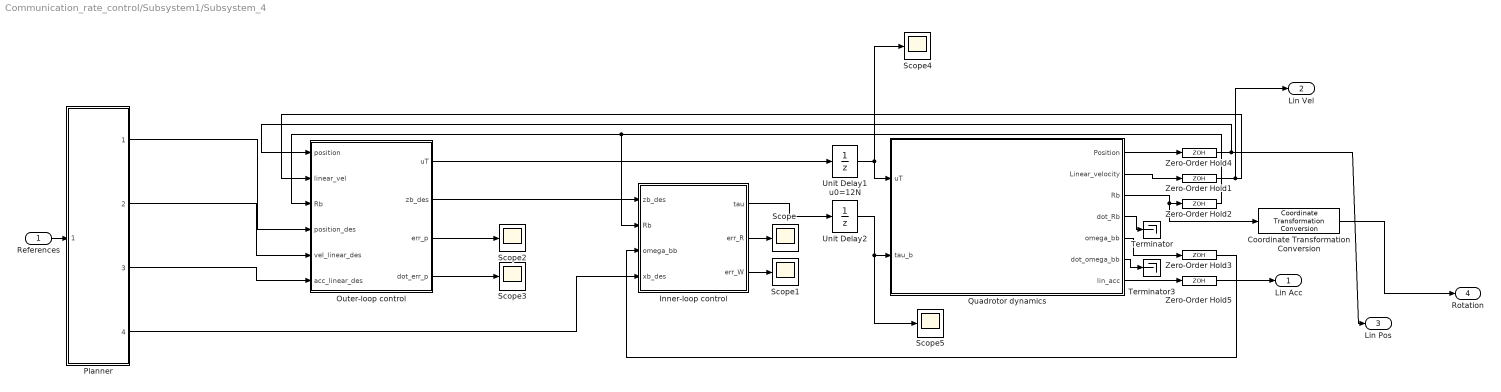
== system Communication_rate_control/Subsystem1/Subsystem_4 ==
  References : Inport
  Coordinate Transformation Conversion : robotcorelib/Coordinate Transformation Conversion  InputRepresentation=Rotation Matrix  InputEulerSequence=ZYX  ShowTrVecInputPort=on  OutputRepresentation=Quaternion  OutputEulerSequence=ZYX  ShowTrVecOutputPort=on  SimulateUsing=Interpreted execution
  Inner-loop control : Subsystem
  Outer-loop control : MATLAB Function  TreatAsAtomicUnit=on
  Planner : Subsystem
  Quadrotor dynamics : Subsystem
  Scope{,1..5} (6 alike) : Scope
      Scope settings: ActiveDisplayYMinimum=-1.2E-5  ActiveDisplayYMaximum=1.2E-5
      Scope1 settings: ActiveDisplayYMinimum=-1.2E-5  ActiveDisplayYMaximum=1.2E-5
      Scope2 settings: ActiveDisplayYMinimum=-3.9E-5  ActiveDisplayYMaximum=1.1E-5  DataLoggingVariableName=ScopeData2
      Scope3 settings: ActiveDisplayYMinimum=-0.00022  ActiveDisplayYMaximum=0.00011  DataLoggingVariableName=ScopeData3
      Scope4 settings: ActiveDisplayYMinimum=11.66748  ActiveDisplayYMaximum=12.03695  DataLoggingVariableName=ScopeData4
      Scope5 settings: ActiveDisplayYMinimum=-0.02035  ActiveDisplayYMaximum=0.02036  DataLoggingVariableName=ScopeData5
  Terminator : Terminator
  Terminator3 : Terminator
  Unit Delay1 u0=12N : UnitDelay  InitialCondition=12  SampleTime=Ts
  Unit Delay2 : UnitDelay  InitialCondition=[0 0 0]  SampleTime=Ts
  Zero-Order Hold{1..5} (5 alike) : ZeroOrderHold  SampleTime=Ts
  Lin Acc : Outport
  Lin Vel : Outport  Port=2
  Lin Pos : Outport  Port=3
  Rotation : Outport  Port=4
  wires:
  Zero-Order Hold5/1 -> Lin Acc/1
  Quadrotor dynamics/7(lin_acc) -> Zero-Order Hold5/1
  Planner/1(position_des) -> Outer-loop control/4(position_des)
  Quadrotor dynamics/1(Position) -> Zero-Order Hold4/1
  Quadrotor dynamics/3(Rb) -> Zero-Order Hold2/1, Coordinate Transformation Conversion/1
  Quadrotor dynamics/4(dot_Rb) -> Terminator/1
  Planner/4(xb_des) -> Inner-loop control/4(xb_des)
  Inner-loop control/1(tau) -> Unit Delay2/1
  Planner/2(linear_velocity_des) -> Outer-loop control/5(vel_linear_des)
  Quadrotor dynamics/2(Linear_velocity) -> Zero-Order Hold1/1
  Quadrotor dynamics/6(dot_omega_bb) -> Terminator3/1
  Outer-loop control/3(err_p) -> Scope2/1
  Coordinate Transformation Conversion/1 -> Rotation/1
  Quadrotor dynamics/5(omega_bb) -> Zero-Order Hold3/1
  Zero-Order Hold2/1 -> Inner-loop control/2(Rb), Outer-loop control/3(Rb)
  References/1 -> Planner/1(References)
  Planner/3(linear_acceleration_des) -> Outer-loop control/6(acc_linear_des)
  Inner-loop control/3(err_W) -> Scope1/1
  Outer-loop control/2(zb_des) -> Inner-loop control/1(zb_des)
  Inner-loop control/2(err_R) -> Scope/1
  Outer-loop control/1(uT) -> Unit Delay1 u0=12N/1
  Unit Delay2/1 -> Quadrotor dynamics/2(tau_b), Scope5/1
  Zero-Order Hold3/1 -> Inner-loop control/3(omega_bb)
  Unit Delay1 u0=12N/1 -> Scope4/1, Quadrotor dynamics/1(uT)
  Outer-loop control/4(dot_err_p) -> Scope3/1
  Zero-Order Hold1/1 -> Outer-loop control/2(linear_vel), Lin Vel/1
  Zero-Order Hold4/1 -> Outer-loop control/1(position), Lin Pos/1
